simulink model "eml_hdl_design_patterns"  (R2026a)
settings: Solver=FixedStepDiscrete  StopTime=10
InitFcn:
  | errMsg  = ['\n\nThis model is only for demonstration purposes.\n\nPlease do not Simulate or code generate directly from this model. \n\nBefore generating code from this model please do copy the relevant blocks of interest from this model to a new model, place them in a subsystem, build a valid test bench around them.\n\nPlease refer to the example model ''eml_hdl_incrementer'' or HDLCoder documentation'];
  | error(sprintf(errMsg));
undefined symbols (not defined in the file or in its folder): C, gain_val, init_val, lower_limit, maxWordLength, thresh, upper_limit
libraries: simulink x2
(part 1 of 5)
settings Model: FPTRunName=Active  ExtModeAutoUpdateStatusClock=off  Creator=The MathWorks, Inc.  LastModifiedBy=The MathWorks, Inc.
settings SolverCC: InsertRTBMode=Auto
settings OptimizationCC: ConditionallyExecuteInputs=off  InitFltsAndDblsToZero=on  EfficientMapNaN2IntZero=off
settings DebuggingCC: AlgebraicLoopMsg=error  UnderspecifiedInitializationDetection=Classic  SingleTaskRateTransMsg=error
settings HardwareCC: ProdHWDeviceType=ASIC/FPGA  ProdEqTarget=off
settings GRTTargetCC: TargetFcnLib=ansi_tfl_tmw_new.mat  CombineOutputUpdateFcns=off  GRTInterface=on

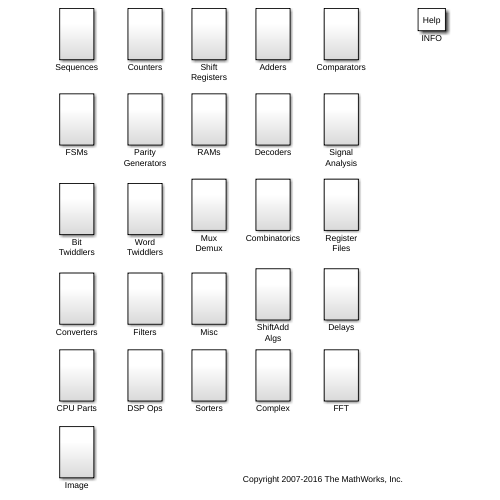
[thumbnail: Simulink's stored preview of the top-level diagram]
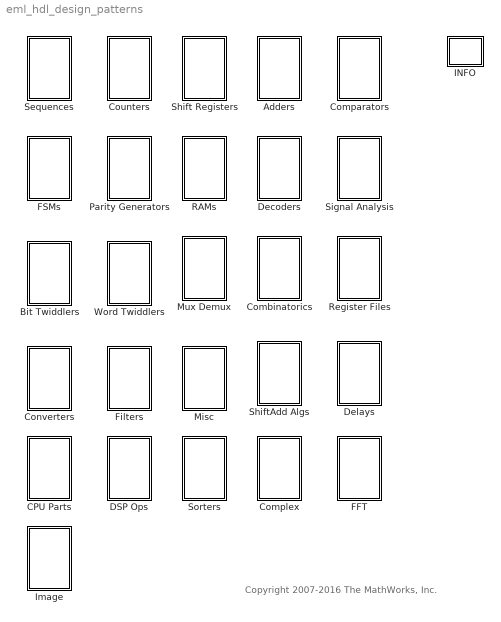
== system eml_hdl_design_patterns ==
  note: Copyright 2007-2016 The MathWorks, Inc.
  Adders : Subsystem
  Bit Twiddlers : Subsystem
  CPU Parts : Subsystem
  Combinatorics : Subsystem
  Comparators : Subsystem
  Complex : Subsystem
  Converters : Subsystem
  Counters : Subsystem
  DSP Ops : Subsystem
  Decoders : Subsystem
  Delays : Subsystem
  FFT : Subsystem
  FSMs : Subsystem
  Filters : Subsystem
  INFO : Subsystem
      settings: OpenFcn=helpview(fullfile (docroot,'toolbox','hdlcoder','ug','hdlcoder_ug.map'), 'slhdlcoder_eml_design_patterns');
      mask Display: disp('Help')
  Image : Subsystem
  Misc : Subsystem
  Mux Demux : Subsystem
  Parity Generators : Subsystem
  RAMs : Subsystem
  Register Files : Subsystem
  Sequences : Subsystem
  Shift Registers : Subsystem
  ShiftAdd Algs : Subsystem
  Signal Analysis : Subsystem
  Sorters : Subsystem
  Word Twiddlers : Subsystem

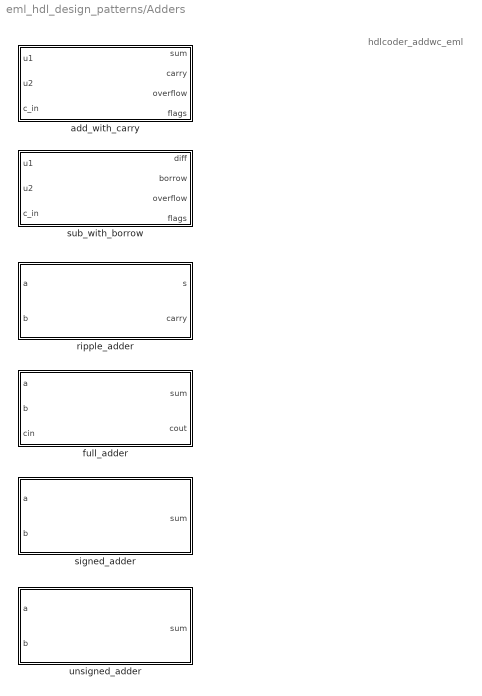
== system eml_hdl_design_patterns/Adders ==
  note: hdlcoder_addwc_eml
  add_with_carry : MATLAB Function  TreatAsAtomicUnit=on
  full_adder : MATLAB Function  TreatAsAtomicUnit=on
  ripple_adder : MATLAB Function  TreatAsAtomicUnit=on
  signed_adder : MATLAB Function  TreatAsAtomicUnit=on
  sub_with_borrow : MATLAB Function  TreatAsAtomicUnit=on
  unsigned_adder : MATLAB Function  TreatAsAtomicUnit=on

== system eml_hdl_design_patterns/Bit Twiddlers ==
  note: hdlcoder_bitops_eml
  note: hdlcoder_int2bits_bits2int
  hdl_bit_ops : MATLAB Function  TreatAsAtomicUnit=on

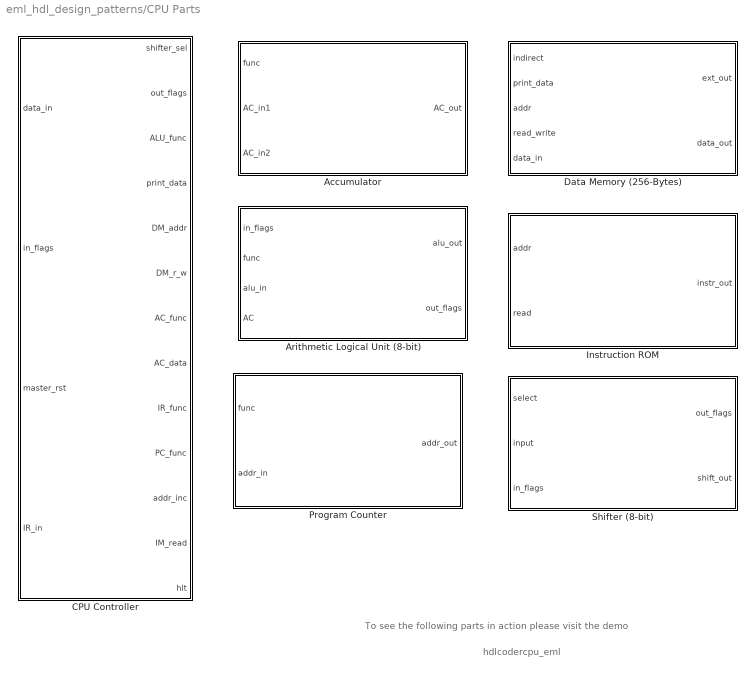
== system eml_hdl_design_patterns/CPU Parts ==
  note: To see the following parts in action please visit the demo
  note: hdlcodercpu_eml
  Accumulator : MATLAB Function  TreatAsAtomicUnit=on
  Arithmetic Logical Unit (8-bit) : MATLAB Function  TreatAsAtomicUnit=on
  CPU Controller : MATLAB Function  TreatAsAtomicUnit=on
  Data Memory (256-Bytes) : MATLAB Function  TreatAsAtomicUnit=on
  Instruction ROM : MATLAB Function  TreatAsAtomicUnit=on
  Program Counter : MATLAB Function  TreatAsAtomicUnit=on
  Shifter (8-bit) : MATLAB Function  TreatAsAtomicUnit=on

== system eml_hdl_design_patterns/Combinatorics ==
  count_ones_blk : MATLAB Function  TreatAsAtomicUnit=on
  eml_expr : MATLAB Function  TreatAsAtomicUnit=on
  hierarchical_mimoparts : Subsystem
  monolithic_mimoparts : MATLAB Function  TreatAsAtomicUnit=on
  pow2Test : MATLAB Function  TreatAsAtomicUnit=on

== system eml_hdl_design_patterns/Comparators ==
  eml_linear_min : MATLAB Function  TreatAsAtomicUnit=on
  eml_tree_min : MATLAB Function  TreatAsAtomicUnit=on

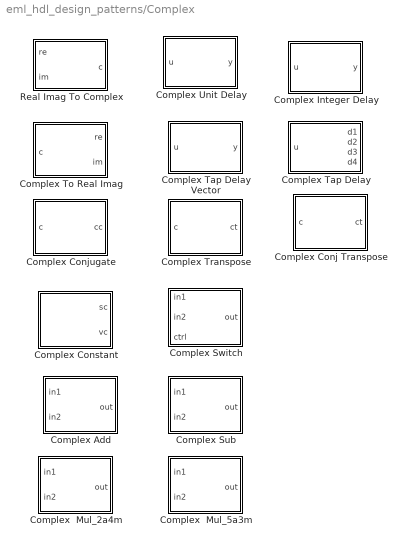
== system eml_hdl_design_patterns/Complex ==
  Complex  Mul_2a4m : MATLAB Function  TreatAsAtomicUnit=on
  Complex  Mul_5a3m : MATLAB Function  TreatAsAtomicUnit=on
  Complex Add : MATLAB Function  TreatAsAtomicUnit=on
  Complex Conj Transpose : MATLAB Function  TreatAsAtomicUnit=on
  Complex Conjugate : MATLAB Function  TreatAsAtomicUnit=on
  Complex Constant : MATLAB Function  TreatAsAtomicUnit=on
  Complex Integer Delay : MATLAB Function  TreatAsAtomicUnit=on
  Complex Sub : MATLAB Function  TreatAsAtomicUnit=on
  Complex Switch : MATLAB Function  TreatAsAtomicUnit=on
  Complex Tap Delay : MATLAB Function  TreatAsAtomicUnit=on
  Complex Tap Delay Vector : MATLAB Function  TreatAsAtomicUnit=on
  Complex To Real Imag : MATLAB Function  TreatAsAtomicUnit=on
  Complex Transpose : MATLAB Function  TreatAsAtomicUnit=on
  Complex Unit Delay : MATLAB Function  TreatAsAtomicUnit=on
  Real Imag To Complex : MATLAB Function  TreatAsAtomicUnit=on

== system eml_hdl_design_patterns/Converters ==
  gray2bin_blk : MATLAB Function  TreatAsAtomicUnit=on

== system eml_hdl_design_patterns/Counters ==
  note: hdlcoder_counters_eml
  counter_clear : MATLAB Function  TreatAsAtomicUnit=on
  counter_mod3 : MATLAB Function  TreatAsAtomicUnit=on
  counter_preset_clear : MATLAB Function  TreatAsAtomicUnit=on
  counter_up_down_enable : MATLAB Function  TreatAsAtomicUnit=on
  gray_counter : MATLAB Function  TreatAsAtomicUnit=on
  johnson_counter : MATLAB Function  TreatAsAtomicUnit=on

== system eml_hdl_design_patterns/DSP Ops ==
  dsp_fold : MATLAB Function  TreatAsAtomicUnit=on
  dsp_scale : MATLAB Function  TreatAsAtomicUnit=on
  dsp_shift : MATLAB Function  TreatAsAtomicUnit=on
  dsp_sum : MATLAB Function  TreatAsAtomicUnit=on

== system eml_hdl_design_patterns/Decoders ==
  note: hdlcoderviterbi2
  note: To see the following parts in action please visit the demo
  decoder_2_by_4 : MATLAB Function  TreatAsAtomicUnit=on
  decoder_n_bit : MATLAB Function  TreatAsAtomicUnit=on
  hierarchical_viterbi : Subsystem
      mask Display: disp('Fixed Point\nViterbi Decoder\nUsing Multiple\nMATLAB Function Blocks');
  monlithic_viterbi : MATLAB Function  TreatAsAtomicUnit=on

== system eml_hdl_design_patterns/Delays ==
  note: hdlcoder_delays_eml
  Integer Delay : MATLAB Function  TreatAsAtomicUnit=on
  Tap Delay : MATLAB Function  TreatAsAtomicUnit=on
  Tap Delay Vector : MATLAB Function  TreatAsAtomicUnit=on
  Unit Delay : MATLAB Function  TreatAsAtomicUnit=on

== system eml_hdl_design_patterns/FFT ==
  note: hdlcoder_fft32_eml
  note: hdlcoder_ofdm_fft_eml
  fft_blk : MATLAB Function  TreatAsAtomicUnit=on

== system eml_hdl_design_patterns/FSMs ==
  note: hdlcoder_fsm_eml
  detect even 1's and odd 0's : MATLAB Function  TreatAsAtomicUnit=on
  mealy_fsm : MATLAB Function  TreatAsAtomicUnit=on
  moore_fsm : MATLAB Function  TreatAsAtomicUnit=on

== system eml_hdl_design_patterns/Filters ==
  lms : MATLAB Function  TreatAsAtomicUnit=on
  sfir_pipelined : MATLAB Function  TreatAsAtomicUnit=on
  symmetric_fir : MATLAB Function  TreatAsAtomicUnit=on

== system eml_hdl_design_patterns/INFO ==
  note: Double Click on the subsystem
      | marked "Help" at the top level
      | to go to the doc page for this model
  note: This model is only for demonstration purposes.
      |
      | It illustrates the power of MATLAB Function Block
      | support in HDLCoder.
      |
      | It shows how to concisely represent common algorithmic
      | operations in ASIC/FPGA applications.
      |
      | Before simulating or code generating from this
      | please copy the relevant blocks from this model to
      | a new model, place them in a subsystem, build
      | a test bench around them with valid inputs.

== system eml_hdl_design_patterns/Image ==
  sobel_edge_behavioral : MATLAB Function  TreatAsAtomicUnit=on
  sobel_edge_serial_pipelined : MATLAB Function  TreatAsAtomicUnit=on
  sobel_edge_serial_pipelined_RAM_mapped : MATLAB Function  TreatAsAtomicUnit=on

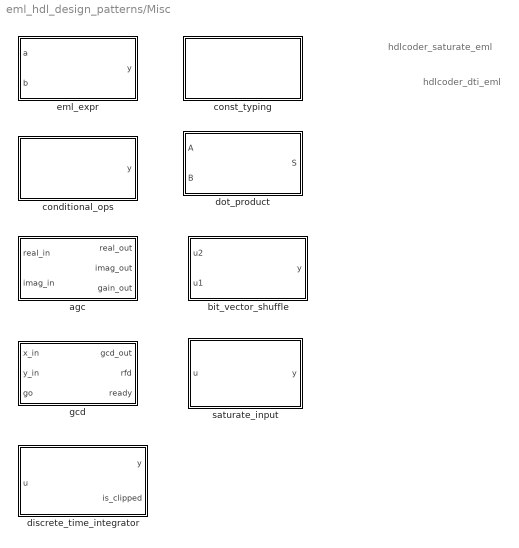
== system eml_hdl_design_patterns/Misc ==
  note: hdlcoder_saturate_eml
  note: hdlcoder_dti_eml
  agc : MATLAB Function  TreatAsAtomicUnit=on
  bit_vector_shuffle : MATLAB Function  TreatAsAtomicUnit=on
  conditional_ops : MATLAB Function  TreatAsAtomicUnit=on
  const_typing : Subsystem
  discrete_time_integrator : MATLAB Function  TreatAsAtomicUnit=on
  dot_product : MATLAB Function  TreatAsAtomicUnit=on
  eml_expr : MATLAB Function  TreatAsAtomicUnit=on
  gcd : MATLAB Function  TreatAsAtomicUnit=on
  saturate_input : MATLAB Function  TreatAsAtomicUnit=on

== system eml_hdl_design_patterns/Mux Demux ==
  demux_using_for_blk : MATLAB Function  TreatAsAtomicUnit=on

== system eml_hdl_design_patterns/Parity Generators ==
  xor_parity_blk : MATLAB Function  TreatAsAtomicUnit=on

== system eml_hdl_design_patterns/RAMs ==
  line_buffer_RAM : MATLAB Function  TreatAsAtomicUnit=on
  sobel_edge_serial_pipelined_RAM_mapped : MATLAB Function  TreatAsAtomicUnit=on

== system eml_hdl_design_patterns/Register Files ==
  dualport_regfile : MATLAB Function  TreatAsAtomicUnit=on
  singleport_regfile : MATLAB Function  TreatAsAtomicUnit=on
  triport_regfile : MATLAB Function  TreatAsAtomicUnit=on

== system eml_hdl_design_patterns/Sequences ==
  stepseq : MATLAB Function  TreatAsAtomicUnit=on

== system eml_hdl_design_patterns/Shift Registers ==
  shift_reg_1by32 : MATLAB Function  TreatAsAtomicUnit=on
  shift_reg_1by64 : MATLAB Function  TreatAsAtomicUnit=on
  shift_reg_universal : MATLAB Function  TreatAsAtomicUnit=on

== system eml_hdl_design_patterns/ShiftAdd Algs ==
  note: hdlcordic_eml
  cordic : Subsystem

== system eml_hdl_design_patterns/Signal Analysis ==
  conv_input_side : MATLAB Function  TreatAsAtomicUnit=on
  conv_output_side : MATLAB Function  TreatAsAtomicUnit=on

== system eml_hdl_design_patterns/Sorters ==
  bitonic_sort : MATLAB Function  TreatAsAtomicUnit=on
  bubble_sort : MATLAB Function  TreatAsAtomicUnit=on

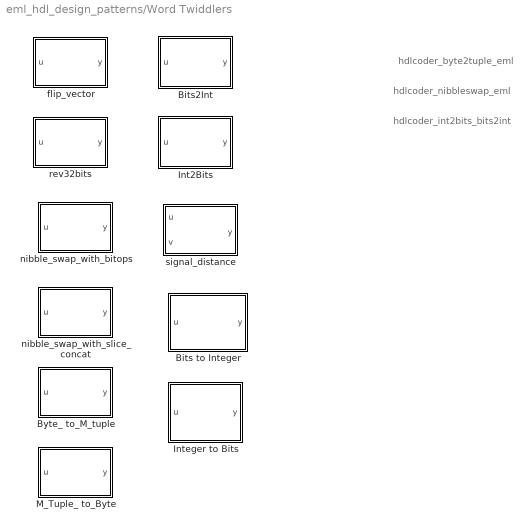
== system eml_hdl_design_patterns/Word Twiddlers ==
  note: hdlcoder_byte2tuple_eml
  note: hdlcoder_nibbleswap_eml
  note: hdlcoder_int2bits_bits2int
  Bits to Integer : MATLAB Function  TreatAsAtomicUnit=on
  Bits2Int : MATLAB Function  TreatAsAtomicUnit=on
  Byte_ to_M_tuple : MATLAB Function  TreatAsAtomicUnit=on
  Int2Bits : MATLAB Function  TreatAsAtomicUnit=on
  Integer to Bits : Subsystem  mask{maxWordLength=maxWordLength}
      mask prompts: maxWordLength "Maximum Word Length"
      mask Display: disp('Integer to Bits')
  M_Tuple_ to_Byte : MATLAB Function  TreatAsAtomicUnit=on
  flip_vector : MATLAB Function  TreatAsAtomicUnit=on
  nibble_swap_with_bitops : MATLAB Function  TreatAsAtomicUnit=on
  nibble_swap_with_slice_concat : MATLAB Function  TreatAsAtomicUnit=on
  rev32bits : MATLAB Function  TreatAsAtomicUnit=on
  signal_distance : MATLAB Function  TreatAsAtomicUnit=on

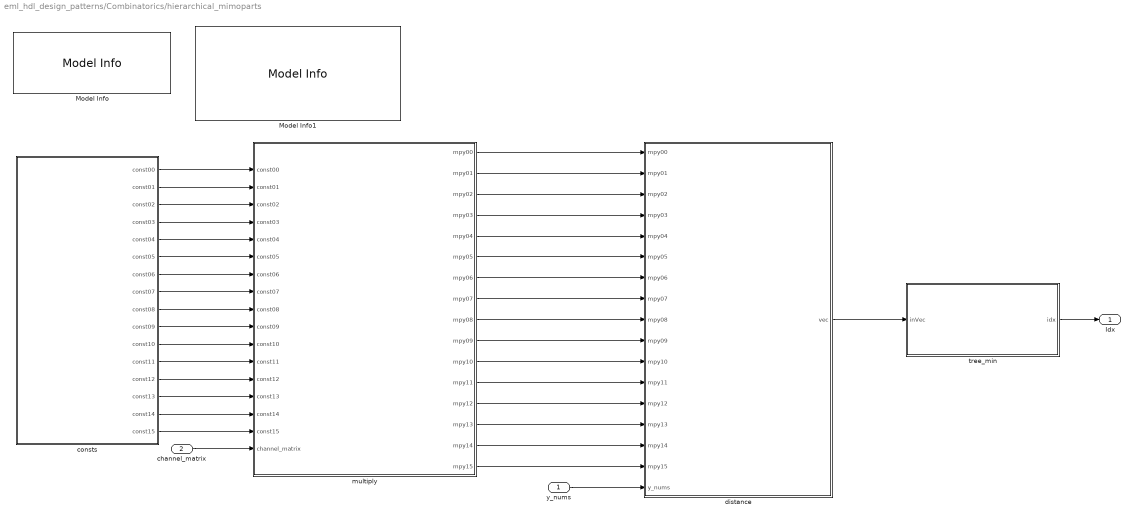
== system eml_hdl_design_patterns/Combinatorics/hierarchical_mimoparts ==
  y_nums : Inport
  channel_matrix : Inport  Port=2
  Model Info : simulink/Model-Wide Utilities/Model Info  Frame=on  DisplayStringWithTags=|  HorizontalTextAlignment=Center  LeftAlignmentValue=0.5
      | This model illustrates some of the
      | key pieces of a MIMO decoder, but
      | is meant only for educational value
      | at this time.
  Model Info1 : simulink/Model-Wide Utilities/Model Info  Frame=on  DisplayStringWithTags=|  HorizontalTextAlignment=Left  LeftAlignmentValue=0.02
      | Key MATLAB Function Block features used in this example:
      | 
      | 1. Creating vector constants
      | 2. Using 'SpecifyPrecision' option in fimath
      | 3. Indexing of vector operands
      | 4. Transpose operations
      | 5. Elementwise product operations
      | 6. Sum of elements operation using sum input
      | 7. Tree min function implementation
      | 8. Vector ports
  consts : MATLAB Function  TreatAsAtomicUnit=on
  distance : MATLAB Function  TreatAsAtomicUnit=on
  multiply : MATLAB Function  TreatAsAtomicUnit=on
  tree_min : MATLAB Function  TreatAsAtomicUnit=on
  Idx : Outport
  wires:
  consts/1(const00) -> multiply/1(const00)
  consts/2(const01) -> multiply/2(const01)
  consts/3(const02) -> multiply/3(const02)
  consts/4(const03) -> multiply/4(const03)
  consts/5(const04) -> multiply/5(const04)
  consts/6(const05) -> multiply/6(const05)
  consts/7(const06) -> multiply/7(const06)
  consts/8(const07) -> multiply/8(const07)
  consts/9(const08) -> multiply/9(const08)
  consts/10(const09) -> multiply/10(const09)
  consts/11(const10) -> multiply/11(const10)
  consts/12(const11) -> multiply/12(const11)
  consts/13(const12) -> multiply/13(const12)
  consts/14(const13) -> multiply/14(const13)
  consts/15(const14) -> multiply/15(const14)
  consts/16(const15) -> multiply/16(const15)
  distance/1(vec) -> tree_min/1(inVec)
  channel_matrix/1 -> multiply/17(channel_matrix)
  multiply/1(mpy00) -> distance/1(mpy00)
  multiply/2(mpy01) -> distance/2(mpy01)
  multiply/3(mpy02) -> distance/3(mpy02)
  multiply/4(mpy03) -> distance/4(mpy03)
  multiply/5(mpy04) -> distance/5(mpy04)
  multiply/6(mpy05) -> distance/6(mpy05)
  multiply/7(mpy06) -> distance/7(mpy06)
  multiply/8(mpy07) -> distance/8(mpy07)
  multiply/9(mpy08) -> distance/9(mpy08)
  multiply/10(mpy09) -> distance/10(mpy09)
  multiply/11(mpy10) -> distance/11(mpy10)
  multiply/12(mpy11) -> distance/12(mpy11)
  multiply/13(mpy12) -> distance/13(mpy12)
  multiply/14(mpy13) -> distance/14(mpy13)
  multiply/15(mpy14) -> distance/15(mpy14)
  multiply/16(mpy15) -> distance/16(mpy15)
  y_nums/1 -> distance/17(y_nums)
  tree_min/1(idx) -> Idx/1

== system eml_hdl_design_patterns/Decoders/hierarchical_viterbi ==
  In1 : Inport  OutDataTypeStr=fixdt(1, 6, 3)  PortDimensions=[2 1]  SampleTime=[10 1]
  BMU1 : MATLAB Function  TreatAsAtomicUnit=on
  PMU1 : Subsystem
  TBU1 : MATLAB Function  TreatAsAtomicUnit=on
  y1 : Outport
  wires:
  TBU1/1(y) -> y1/1
  BMU1/1(bm) -> PMU1/1(bm)
  PMU1/1(dec) -> TBU1/1(dec)
  PMU1/2(index) -> TBU1/2(index)
  In1/1 -> BMU1/1(u)

== system eml_hdl_design_patterns/Misc/const_typing ==
  typed : MATLAB Function  TreatAsAtomicUnit=on
  untyped : MATLAB Function  TreatAsAtomicUnit=on

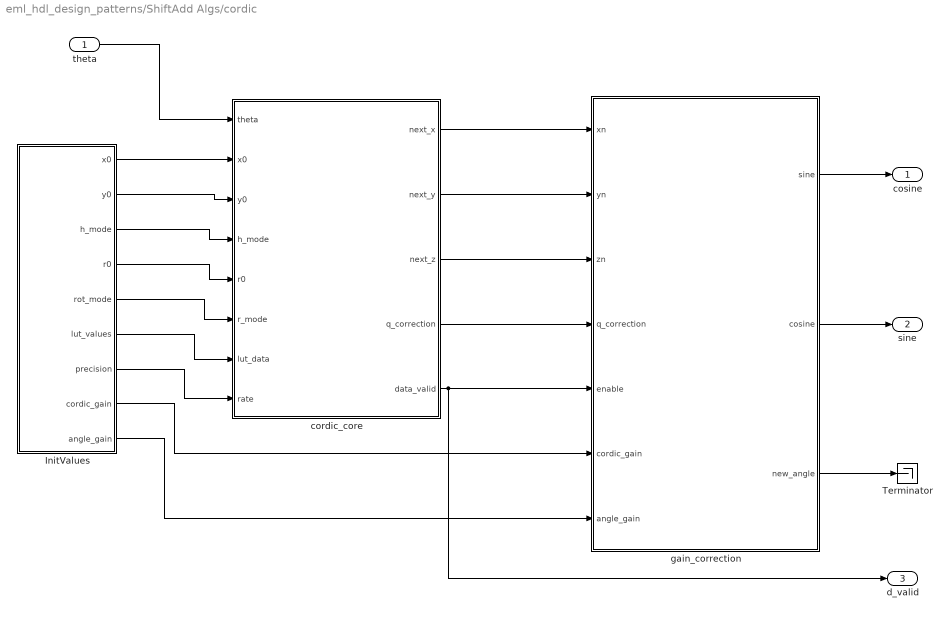
== system eml_hdl_design_patterns/ShiftAdd Algs/cordic ==
  theta : Inport
  InitValues : Subsystem
  Terminator : Terminator
  cordic_core : Subsystem
  gain_correction : MATLAB Function  TreatAsAtomicUnit=on
  cosine : Outport
  sine : Outport  Port=2
  d_valid : Outport  Port=3
  wires:
  gain_correction/1(sine) -> cosine/1
  gain_correction/2(cosine) -> sine/1
  gain_correction/3(new_angle) -> Terminator/1
  cordic_core/1(next_x) -> gain_correction/1(xn)
  cordic_core/2(next_y) -> gain_correction/2(yn)
  cordic_core/3(next_z) -> gain_correction/3(zn)
  cordic_core/4(q_correction) -> gain_correction/4(q_correction)
  cordic_core/5(data_valid) -> gain_correction/5(enable), d_valid/1
  InitValues/8(cordic_gain) -> gain_correction/6(cordic_gain)
  InitValues/9(angle_gain) -> gain_correction/7(angle_gain)
  theta/1 -> cordic_core/1(theta)
  InitValues/1(x0) -> cordic_core/2(x0)
  InitValues/2(y0) -> cordic_core/3(y0)
  InitValues/3(h_mode) -> cordic_core/4(h_mode)
  InitValues/4(r0) -> cordic_core/5(r0)
  InitValues/5(rot_mode) -> cordic_core/6(r_mode)
  InitValues/6(lut_values) -> cordic_core/7(lut_data)
  InitValues/7(precision) -> cordic_core/8(rate)

== system eml_hdl_design_patterns/Word Twiddlers/Integer to Bits ==
  u : Inport
  MATLAB Function : MATLAB Function  TreatAsAtomicUnit=on
  y : Outport
  wires:
  MATLAB Function/1(y) -> y/1
  u/1 -> MATLAB Function/1(u)

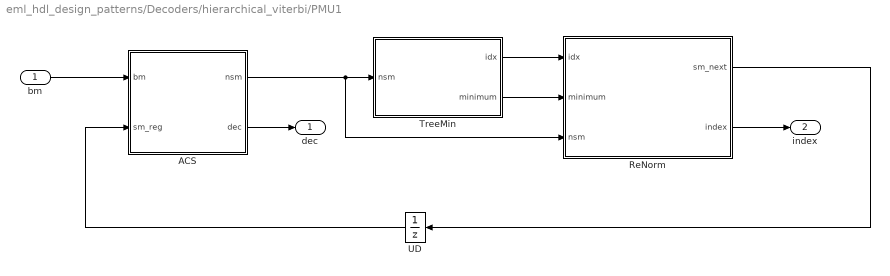
== system eml_hdl_design_patterns/Decoders/hierarchical_viterbi/PMU1 ==
  bm : Inport
  ACS : MATLAB Function  TreatAsAtomicUnit=on
  ReNorm : MATLAB Function  TreatAsAtomicUnit=on
  TreeMin : MATLAB Function  TreatAsAtomicUnit=on
  UD : UnitDelay  SampleTime=-1
  dec : Outport
  index : Outport  Port=2
  wires:
  bm/1 -> ACS/1(bm)
  ACS/1(nsm) -> TreeMin/1(nsm), ReNorm/3(nsm)
  TreeMin/1(idx) -> ReNorm/1(idx)
  TreeMin/2(minimum) -> ReNorm/2(minimum)
  ACS/2(dec) -> dec/1
  ReNorm/1(sm_next) -> UD/1
  ReNorm/2(index) -> index/1
  UD/1 -> ACS/2(sm_reg)

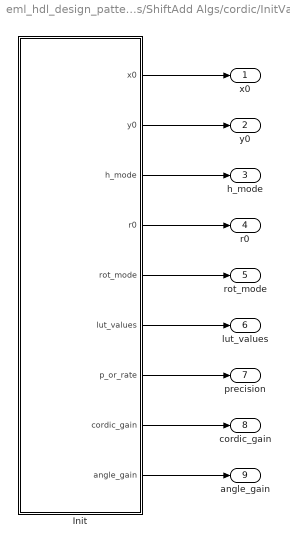
== system eml_hdl_design_patterns/ShiftAdd Algs/cordic/InitValues ==
  Init : MATLAB Function  TreatAsAtomicUnit=on
  x0 : Outport
  y0 : Outport  Port=2
  h_mode : Outport  Port=3
  r0 : Outport  Port=4
  rot_mode : Outport  Port=5
  lut_values : Outport  Port=6
  precision : Outport  Port=7
  cordic_gain : Outport  Port=8
  angle_gain : Outport  Port=9
  wires:
  Init/1(x0) -> x0/1
  Init/2(y0) -> y0/1
  Init/3(h_mode) -> h_mode/1
  Init/4(r0) -> r0/1
  Init/5(rot_mode) -> rot_mode/1
  Init/6(lut_values) -> lut_values/1
  Init/7(p_or_rate) -> precision/1
  Init/8(cordic_gain) -> cordic_gain/1
  Init/9(angle_gain) -> angle_gain/1

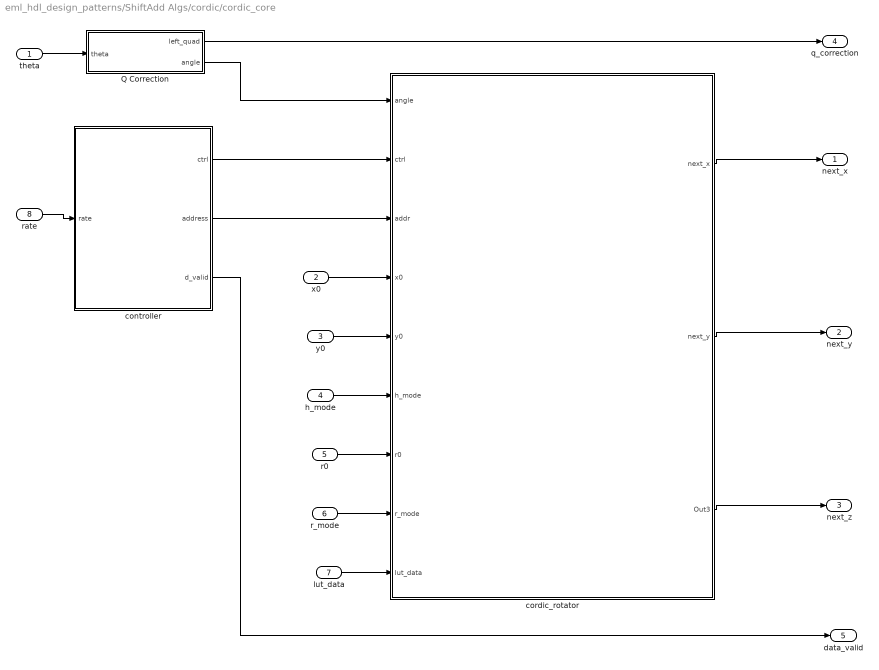
== system eml_hdl_design_patterns/ShiftAdd Algs/cordic/cordic_core ==
  theta : Inport
  x0 : Inport  Port=2
  y0 : Inport  Port=3
  h_mode : Inport  Port=4
  r0 : Inport  Port=5
  r_mode : Inport  Port=6
  lut_data : Inport  Port=7
  rate : Inport  Port=8
  Q Correction : MATLAB Function  TreatAsAtomicUnit=on
  controller : MATLAB Function  TreatAsAtomicUnit=on
  cordic_rotator : Subsystem
  next_x : Outport
  next_y : Outport  Port=2
  next_z : Outport  Port=3
  q_correction : Outport  Port=4
  data_valid : Outport  Port=5
  wires:
  controller/3(d_valid) -> data_valid/1
  rate/1 -> controller/1(rate)
  cordic_rotator/2(next_y) -> next_y/1
  cordic_rotator/1(next_x) -> next_x/1
  cordic_rotator/3(Out3) -> next_z/1
  theta/1 -> Q Correction/1(theta)
  Q Correction/1(left_quad) -> q_correction/1
  x0/1 -> cordic_rotator/4(x0)
  h_mode/1 -> cordic_rotator/6(h_mode)
  r0/1 -> cordic_rotator/7(r0)
  r_mode/1 -> cordic_rotator/8(r_mode)
  lut_data/1 -> cordic_rotator/9(lut_data)
  y0/1 -> cordic_rotator/5(y0)
  Q Correction/2(angle) -> cordic_rotator/1(angle)
  controller/1(ctrl) -> cordic_rotator/2(ctrl)
  controller/2(address) -> cordic_rotator/3(addr)

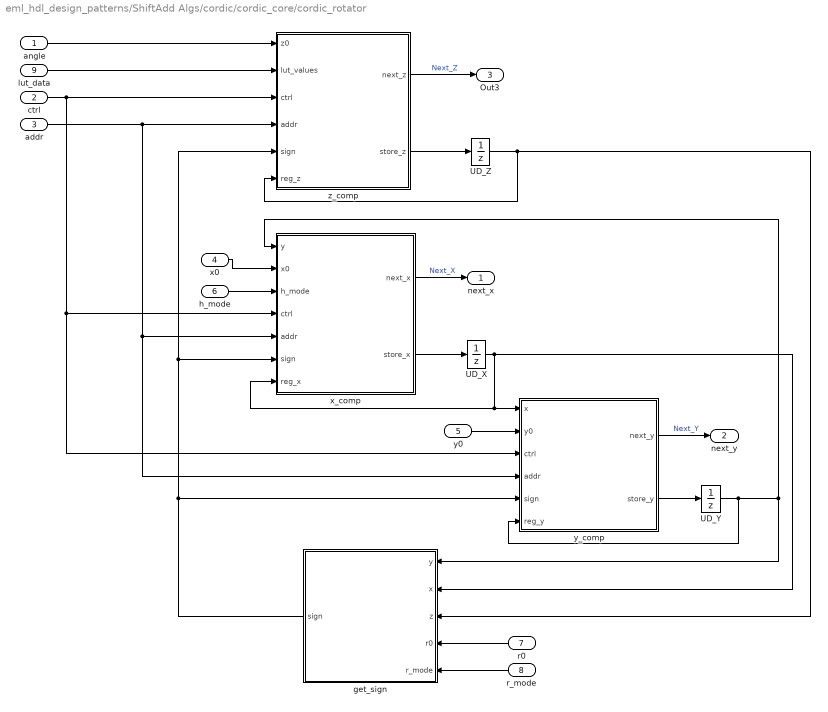
== system eml_hdl_design_patterns/ShiftAdd Algs/cordic/cordic_core/cordic_rotator ==
  angle : Inport
  ctrl : Inport  Port=2
  addr : Inport  Port=3
  x0 : Inport  Port=4
  y0 : Inport  Port=5
  h_mode : Inport  Port=6
  r0 : Inport  Port=7
  r_mode : Inport  Port=8
  lut_data : Inport  Port=9
  UD_X : UnitDelay  SampleTime=-1
  UD_Y : UnitDelay  SampleTime=-1
  UD_Z : UnitDelay  SampleTime=-1
  get_sign : MATLAB Function  TreatAsAtomicUnit=on
  x_comp : MATLAB Function  TreatAsAtomicUnit=on
  y_comp : MATLAB Function  TreatAsAtomicUnit=on
  z_comp : MATLAB Function  TreatAsAtomicUnit=on
  next_x : Outport
  next_y : Outport  Port=2
  Out3 : Outport  Port=3
  wires:
  r_mode/1 -> get_sign/5(r_mode)
  r0/1 -> get_sign/4(r0)
  addr/1 -> y_comp/4(addr), x_comp/5(addr), z_comp/4(addr)
  ctrl/1 -> y_comp/3(ctrl), x_comp/4(ctrl), z_comp/3(ctrl)
  lut_data/1 -> z_comp/2(lut_values)
  y0/1 -> y_comp/2(y0)
  h_mode/1 -> x_comp/3(h_mode)
  x0/1 -> x_comp/2(x0)
  y_comp/2(store_y) -> UD_Y/1
  get_sign/1(sign) -> y_comp/5(sign), z_comp/5(sign), x_comp/6(sign)
  UD_Z/1 -> z_comp/6(reg_z), get_sign/3(z)
  UD_Y/1 -> y_comp/6(reg_y), get_sign/1(y), x_comp/1(y)
  UD_X/1 -> y_comp/1(x), x_comp/7(reg_x), get_sign/2(x)
  x_comp/2(store_x) -> UD_X/1
  z_comp/2(store_z) -> UD_Z/1
  angle/1 -> z_comp/1(z0)
  x_comp/1(next_x) -> next_x/1  "Next_X"
  y_comp/1(next_y) -> next_y/1  "Next_Y"
  z_comp/1(next_z) -> Out3/1  "Next_Z"

== matlab function eml_hdl_design_patterns/Complex/Complex  Mul_2a4m ==
  settings: fimath=|
      | fimath(...
      | 'RoundMode', 'floor',...
      | 'OverflowMode', 'wrap',...
      | 'ProductMode', 'FullPrecision', 'ProductWordLength', 32,...
      | 'SumMode', 'FullPrecision', 'SumWordLength', 32,...
      | 'CastBeforeSum', true)
  data: out output; in1 input fixdt(1,14,2); in2 input fixdt(1,14,2)
function out = fcn(in1, in2)
% Compute Multiply
%
%  out_re = in1_re * in2_re - in1_im * in2_im
%  out_im = in1_re * in2_im + in1_im * in2_re
%
% For fixed point inputs 'SumMode' and 'ProductMode' options on the 
% block fimath decides the sum and product semantics in the above equations. 
%
% In this example SumMode and ProductMode are set to FullPrecision 
% which is optimal for HDLCodegen
%
% The default complex multiplication operator uses 2adders and 4multipliers
% shown in the above equations.


f = fimath(in1);
nt = numerictype(in1);

out = fi(in1*in2, nt, f);

== matlab function eml_hdl_design_patterns/Complex/Complex  Mul_5a3m ==
  settings: fimath=|
      | fimath(...
      | 'RoundMode', 'floor',...
      | 'OverflowMode', 'wrap',...
      | 'ProductMode', 'FullPrecision', 'ProductWordLength', 32,...
      | 'SumMode', 'FullPrecision', 'SumWordLength', 32,...
      | 'CastBeforeSum', true)
  data: out output; in1 input; in2 input
function out = fcn(in1, in2)
% Compute Complex Multiply
% 
% The canonical definition of complex multiplication is:
%
%  out_re = in1_re * in2_re - in1_im * in2_im
%  out_im = in1_re * in2_im + in1_im * in2_re
%
% This definition uses 2 adders and 4 multipliers, as shown above.
%
% However, algebraic manipiulation of these equations results in another pair of
% equations that requires only 3 multipliers, while requiring 5 adders. This
% tradeoff results in reduced area consumption for complex multiplication.
%
%  (a + bi) * (c + di) ==> e + fi
%
%    where
%
%  e = (a + b)*(c - d) - b*c + a*d
%  f = b*c + a*d
%
% For fixed point inputs, the 'SumMode' and 'ProductMode' options on the 
% block fimath decide the sum and product semantics for fixed point calculations.
%
% In this example, SumMode and ProductMode are set to FullPrecision, which is
% optimal for HDL code generation.

fm = fimath(in1);
nt = numerictype(in1);

a = real(in1);
b = imag(in1);

c = real(in2);
d = imag(in2);

bc = fi(b .* c, nt, fm);
ad = fi(a .* d, nt, fm);

% Compute the real part
e = fi((a + b) .* (c - d) - bc + ad, nt, fm);
% Compute the imaginary part
f = fi(bc + ad, nt, fm);

out = complex(e, f);
end

== matlab function eml_hdl_design_patterns/Delays/Integer Delay ==
  settings: fimath=|
      | fimath(...
      | 'RoundMode', 'floor',...
      | 'OverflowMode', 'wrap',...
      | 'ProductMode', 'FullPrecision', 'ProductWordLength', 32,...
      | 'SumMode', 'FullPrecision', 'SumWordLength', 32,...
      | 'CastBeforeSum', true)
  data: u input; y output; N parameter
function y = fcn(u, N)

% The Integer Delay block delays its input by N sample periods. 
% The block accepts one input and generates one output, both of which
% can be scalar or vector. If the input is a vector, all elements of the 
% vector are delayed by the same sample period.

% In this example N is hardwired as 4; This function behaves as Integer 
% delay block and delays inputs by 4 sample hits.

persistent u_d;
if isempty(u_d)
	% defines initial value driven by integer delay 
    % from time step 0 to time step N-1
    u_d = fi(zeros(1,N), numerictype(u), fimath(u));
end

y = u_d(N);

u_d = [u, u_d(1:N-1)];

== matlab function eml_hdl_design_patterns/Counters/johnson_counter ==
  settings: fimath=|
      | fimath(...
      | 'RoundMode', 'floor',...
      | 'OverflowMode', 'saturate',...
      | 'ProductMode', 'FullPrecision', 'ProductWordLength', 32,...
      | 'SumMode', 'FullPrecision', 'SumWordLength', 32,...
      | 'CastBeforeSum', true)
  data: enable input boolean; count output fixdt(0,4,0) size=1
function count = fcn(enable)

% A johnson counter is a circular shift register that feeds the LSB with
% the inverted MSB.  It generates a pattern like
% 0000
% 0001
% 0011
% 0111
% 1111
% 1110
% 1100
% 1000
% 0000
% 0001

% This counter is configured to rollover.  If this is not desirable,
% set result_fm 'OverflowMode' to 'saturate'.

result_nt = numerictype(0,4,0);
result_fm = fimath('OverflowMode', 'wrap', 'RoundMode', 'floor');

persistent count_reg;

if isempty(count_reg)
    count_reg = fi(0, result_nt, result_fm);
end

% Assign the output even when we're not enabled.
count = count_reg;

if enable
   oldmsb = getmsb(count_reg);
   count_reg = bitsll(count_reg, 1);   
   count_reg = bitset(count_reg, 1, ~uint8(oldmsb));
end

== matlab function eml_hdl_design_patterns/Delays/Tap Delay Vector ==
  settings: fimath=|
      | fimath(...
      | 'RoundMode', 'floor',...
      | 'OverflowMode', 'wrap',...
      | 'ProductMode', 'FullPrecision', 'ProductWordLength', 32,...
      | 'SumMode', 'FullPrecision', 'SumWordLength', 32,...
      | 'CastBeforeSum', true)
  data: u input; y output
function y = fcn(u)
% The Tapped Delay function delays its input by the specified number 
% of sample periods, and outputs all the delayed versions in a vector
% form.

% In this example N is hardwired to 4.

persistent u_d;
if isempty(u_d)
    u_d = fi(zeros(1,4), numerictype(u), fimath(u));
end

y = u_d;

u_d = [u_d(2), u_d(3), u_d(4), u];

== matlab function eml_hdl_design_patterns/Delays/Tap Delay ==
  settings: fimath=|
      | fimath(...
      | 'RoundMode', 'floor',...
      | 'OverflowMode', 'wrap',...
      | 'ProductMode', 'FullPrecision', 'ProductWordLength', 32,...
      | 'SumMode', 'FullPrecision', 'SumWordLength', 32,...
      | 'CastBeforeSum', true)
  data: u input; d1 output; d2 output; d3 output; d4 output
function [d1, d2, d3, d4] = fcn(u)
%The Tapped Delay function delays its input by the specified number 
% of sample periods, and outputs all the delayed versions.

% In this example the number of output taps is hardwired to 4.

persistent u_d;
if isempty(u_d)
    % defines initial value driven by integer delay 
    % from time step 0 to time step N-1
    u_d = fi(zeros(1,4), numerictype(u), fimath(u));
end

d1 = u_d(1);
d2 = u_d(2);
d3 = u_d(3);
d4 = u_d(4);

u_d = [u_d(2:4), u];

== matlab function eml_hdl_design_patterns/Word Twiddlers/Int2Bits ==
  data: u input; y output
function y = fcn(u)
% Converts Integer(8bits) to a 1-D array Bits

y = bitget(u, [8:-1:1])';

== matlab function eml_hdl_design_patterns/Image/sobel_edge_serial_pipelined ==
  settings: fimath=|
      | fimath(...
      | 'RoundMode', 'floor',...
      | 'OverflowMode', 'wrap',...
      | 'ProductMode', 'FullPrecision', 'ProductWordLength', 32,...
      | 'SumMode', 'FullPrecision', 'SumWordLength', 32,...
      | 'CastBeforeSum', true)
  data: u input fixdt(1,9,0); e output; thresh parameter uint8
function e = fcn(u, thresh)
% Pipelined Sobel Edge Detection algorithm on serialized image.

[xfo, yfo] =  filter(u);
xfd = filterdelay12(xfo);
yfd = filterdelay13(yfo);
ax = abs(xfd);
ay = abs(yfd);
t = (ax + ay >= thresh);
e = filterdelay14(t);

end

%%%%%%%%%%%%%%%%%%%%%%%%%%%%%%%%%%%%%%%%%%%%%%%%%%%%%%%%%%%%%%%%%%%%%%%%%%%
% Compute convolution of serialized image data with sobel masks
%%%%%%%%%%%%%%%%%%%%%%%%%%%%%%%%%%%%%%%%%%%%%%%%%%%%%%%%%%%%%%%%%%%%%%%%%%%
function [xfo, yfo] =  filter(u)

lb1 = line_buffer1(u);
lb2 = line_buffer2(lb1);

ud1 = filterdelay1(u);
ud2 = filterdelay2(ud1);

lb1d1 = filterdelay3(lb1);
lb1d2 = filterdelay4(lb1d1);

lb2d1 = filterdelay5(lb2);
lb2d2 = filterdelay6(lb2d1);

xfo = xf(u, ud1, ud2, lb2, lb2d1, lb2d2);
yfo = yf(ud2, u, lb1d2, lb1, lb2d2, lb2);

end

%%%%%%%%%%%%%%%%%%%%%%%%%%%%%%%%%%%%%%%%%%%%%%%%%%%%%%%%%%%%%%%%%%%%%%%%%%%
% Compute x gradient
%%%%%%%%%%%%%%%%%%%%%%%%%%%%%%%%%%%%%%%%%%%%%%%%%%%%%%%%%%%%%%%%%%%%%%%%%%%
function xf_out = xf(u, xd1, xd2, lb2, zd1, zd2)
c2 = fi(2, 1,3,0, fimath(u));

t1 = fi(xd1 * c2, 1,10,0, fimath(u));
a1 = fi(u + t1 + xd2, 1,11,0, fimath(u));
pa1 = filterdelay7(a1);

t1 = fi(zd1 * c2, 1,10,0, fimath(u));
a2 = fi(lb2 + t1 + zd2, 1,11,0, fimath(u));
pa2 = filterdelay8(a2);

xf_out = fi(pa1 - pa2, 1,12,0, fimath(u));

end

%%%%%%%%%%%%%%%%%%%%%%%%%%%%%%%%%%%%%%%%%%%%%%%%%%%%%%%%%%%%%%%%%%%%%%%%%%%
% Compute y gradient
%%%%%%%%%%%%%%%%%%%%%%%%%%%%%%%%%%%%%%%%%%%%%%%%%%%%%%%%%%%%%%%%%%%%%%%%%%%
function yf_out = yf(xd2, u, yd2, lb1, zd2, lb2)
t = fi(xd2 - u, 1,11,0, fimath(u));
pa1 = filterdelay9(t);

t = fi(yd2 - lb1, 1,11,0, fimath(u));
c2 = fi(2, 1,3,0, fimath(u));
a2 = fi(c2 * t, 1,11,0, fimath(u));
pa2 = filterdelay10(a2);

t = fi(zd2 - lb2, 1,11,0, fimath(u));
pa3 = filterdelay11(t);

yf_out = fi(pa1 + pa2 + pa3, 1,13,0, fimath(u));

end

%%%%%%%%%%%%%%%%%%%%%%%%%%%%%%%%%%%%%%%%%%%%%%%%%%%%%%%%%%%%%%%%%%%%%%%%%%%
% Line Buffers %
%%%%%%%%%%%%%%%%%%%%%%%%%%%%%%%%%%%%%%%%%%%%%%%%%%%%%%%%%%%%%%%%%%%%%%%%%%%
function y = line_buffer1(u)
N = 100;
persistent u_d;
if isempty(u_d)
    u_d = fi(zeros(1,N), numerictype(u), fimath(u));
end

y = u_d(N);
u_d = [u, u_d(1:N-1)];
end

function y = line_buffer2(u)
N = 100;
persistent u_d;
if isempty(u_d)
    u_d = fi(zeros(1,N), numerictype(u), fimath(u));
end

y = u_d(N);
u_d = [u, u_d(1:N-1)];
end


%%%%%%%%%%%%%%%%%%%%%%%%%%%%%%%%%%%%%%%%%%%%%%%%%%%%%%%%%%%%%%%%%%%%%%%%%%%
% Filter Delays %
%%%%%%%%%%%%%%%%%%%%%%%%%%%%%%%%%%%%%%%%%%%%%%%%%%%%%%%%%%%%%%%%%%%%%%%%%%%

function y = filterdelay1(u)
persistent u_d;
if isempty(u_d)
    u_d = fi(0, numerictype(u), fimath(u));
end
y = u_d;
u_d = u;
end

function y = filterdelay2(u)
persistent u_d;
if isempty(u_d)
    u_d = fi(0, numerictype(u), fimath(u));
end
y = u_d;
u_d = u;
end

function y = filterdelay3(u)
persistent u_d;
if isempty(u_d)
    u_d = fi(0, numerictype(u), fimath(u));
end
y = u_d;
u_d = u;
end

function y = filterdelay4(u)
persistent u_d;
if isempty(u_d)
    u_d = fi(0, numerictype(u), fimath(u));
end
y = u_d;
u_d = u;
end

function y = filterdelay5(u)
persistent u_d;
if isempty(u_d)
    u_d = fi(0, numerictype(u), fimath(u));
end
y = u_d;
u_d = u;
end

function y = filterdelay6(u)
persistent u_d;
if isempty(u_d)
    u_d = fi(0, numerictype(u), fimath(u));
end
y = u_d;
u_d = u;
end

function y = filterdelay7(u)
persistent u_d;
if isempty(u_d)
    u_d = fi(0, numerictype(u), fimath(u));
end
y = u_d;
u_d = u;
end

function y = filterdelay8(u)
persistent u_d;
if isempty(u_d)
    u_d = fi(0, numerictype(u), fimath(u));
end
y = u_d;
u_d = u;
end

function y = filterdelay9(u)
persistent u_d;
if isempty(u_d)
    u_d = fi(0, numerictype(u), fimath(u));
end
y = u_d;
u_d = u;
end

function y = filterdelay10(u)
persistent u_d;
if isempty(u_d)
    u_d = fi(0, numerictype(u), fimath(u));
end
y = u_d;
u_d = u;
end

function y = filterdelay11(u)
persistent u_d;
if isempty(u_d)
    u_d = fi(0, numerictype(u), fimath(u));
end
y = u_d;
u_d = u;
end

function y = filterdelay12(u)
persistent u_d;
if isempty(u_d)
    u_d = fi(0, numerictype(u), fimath(u));
end
y = u_d;
u_d = u;
end

function y = filterdelay13(u)
persistent u_d;
if isempty(u_d)
    u_d = fi(0, numerictype(u), fimath(u));
end
y = u_d;
u_d = u;
end

function y = filterdelay14(u)
persistent u_d;
if isempty(u_d)
    u_d = false;
end
y = u_d;
u_d = u;
end

== matlab function eml_hdl_design_patterns/Filters/lms ==
  settings: fimath=|
      | fimath(...
      | 'RoundMode', 'Nearest',...
      | 'OverflowMode', 'Saturate',...
      | 'ProductMode', 'KeepLSB', 'ProductWordLength', 32, ...
      | 'SumMode', 'KeepLSB', 'SumWordLength', 32, ...
      | 'CastBeforeSum', true)
  data: input input; y output; desired input; step_size input; reset_weights input
function y = fcn(input, desired, step_size, reset_weights)
% Adaptive Noise Canceler algorithm using Least Mean Square (LMS) filter 
% implemented with a MATLAB Function. 
%
% 'input'  : The signal from Exterior Mic which records the ambient noise.
% 'desired': The signal from Pilot's Mic which includes 
%            original music signal and the noise signal
% 'err_sig': The difference between the 'desired' and the filtered 'input'
%            It represents the estimated music signal (output of this block)
% 
% The LMS filter is trying to retrieve the original music signal ('err_sig') 
% from Pilot's Mic by filtering the Exterior Mic's signal and using it to 
% cancel the noise in Pilot's Mic. The coefficients/weights of the filter 
% are updated(adapted) in realtime based on 'input' and 'err_sig'.

fm = fimath(input);

% register filter coefficients
persistent filter_coefficients;
if isempty(filter_coefficients)
    filter_coefficients = fi(zeros(1, 40), 1, 16, 16, fm);
end

% Variable Filter
% call 'tapped_delay_fcn' function on path to create 40-step tapped delay
delayed_signal = tapped_delay_fcn(input);

% apply filter coefficients 
weight_applied = fi(delayed_signal .* filter_coefficients, 1, 32, 20, fm);

% call 'treesum' function on matlab path to sum up the results
filtered_signal = treesum_fcn(weight_applied);

% Output estimated Original Signal
err_sig = fi(desired - filtered_signal, 1, 16, 13, fm);
y = err_sig;

% Update Weights
% call 'update_weight_fcn' function on matlab path to 
% calculate the new weights
updated_weight = update_weight_fcn(step_size, err_sig, delayed_signal, ...
                                   filter_coefficients, reset_weights);

% update filter coefficients register
filter_coefficients = updated_weight;


function tap_delay = tapped_delay_fcn(input)
% The Tapped Delay function delays its input by the specified number 
% of sample periods, and outputs all the delayed versions in a vector
% form. The output includes current input

% NOTE: To instruct MATLAB Coder to compile an external function, 
% add the following compilation directive or pragma to the function code
%#codegen

persistent u_d;
if isempty(u_d)
    u_d = fi(zeros(1,40), numerictype(input), fimath(input));
end


u_d = [u_d(2:40), input];

tap_delay = u_d;


function y = treesum_fcn(u)
%Implement the 'sum' function without a for-loop
%  y = sum(u);

%  The loop based implementation of 'sum' function is not ideal for 
%  HDL generation and results in a longer critical path. 
%  A tree is more efficient as it results in
%  delay of log2(N) instead of a delay of N delay

%  This implementation shows how to explicitly implement the vector sum in 
%  a tree shape to enable hardware optimizations.

%  The ideal way to code this generically for any length of 'u' is to use 
%  recursion but it is not currently supported by the MATLAB Function Block.


% NOTE: To instruct MATLAB Coder to compile an external function, 
% add the following compilation directive or pragma to the function code
%#eml


% Please note that this implementation is hardwired for a 40tap filter.

%20
level1 = vsum(u);

%10
level2 = vsum(level1);

%5
level3 = vsum(level2);

%3
level4 = vsum(level3);

%2
level5 = vsum(level4);

%1
level6 = vsum(level5);


y = level6;



function output = vsum(input)

nt = numerictype(input);
fm = fimath(input);

nd = numel(input)/2;
vt = input(1:2:end);
    
for i = int32(1:nd)
    k = int32(i*2);
    vt(i) = fi(vt(i) + input(k), nt, fm);
end

output = vt;


function weights = update_weight_fcn(step_size, err_sig, delayed_signal, filter_coefficients, reset_weights)
% This function updates the adaptive filter weights based on LMS algorithm

% NOTE: To instruct MATLAB Coder to compile an external function, 
% add the following compilation directive or pragma to the function code
%#eml

fm = fimath(step_size);

step_sig = fi(step_size .* err_sig, 1, 32, 20, fm);
correction_factor = fi(delayed_signal .* step_sig, 1, 32, 20, fm);
updated_weight = fi(correction_factor + filter_coefficients, 1, 16, 16, fm);

if reset_weights
    weights = fi(zeros(1,40), 1, 16, 16, fm);
else    
    weights = updated_weight;
end

== matlab function eml_hdl_design_patterns/Image/sobel_edge_behavioral ==
  data: u input uint8; e output; ref_thresh parameter uint8
function e = fcn(u, ref_thresh)
% SOBEL EDGE DETECTION
%
% Edges characterize boundaries and are therefore a problem of fundamental 
% importance in image processing. Edges in images are areas with strong 
% intensity contrasts. Edge detecting an image significantly 
% reduces the amount of data and filters out useless information, 
% while preserving the important structural properties in an image. 

% The Sobel operator performs a 2-D spatial gradient measurement on an 
% image. Typically it is used to find the approximate absolute gradient 
% magnitude at each point in an input grayscale image. The Sobel edge 
% detector uses a pair of 3x3 convolution masks, one estimating the 
% gradient in the x-direction (columns) and the other estimating the 
% gradient in the y-direction (rows). A convolution mask is usually much 
% smaller than the actual image. As a result, the mask is slid over the 
% image, manipulating a square of pixels at a time. The actual Sobel 
% masks are shown below

% Note that 'gy' is simply 'gx' rotated 90deg anti clockwise
gx = [-1,  0,  1; 
      -2,  0,  2; 
      -1,  0,  1];
  
gy = [ 1,  2,  1;  
       0,  0,  0; 
      -1, -2, -1];

a1t = abs(conv2(gx, double(u), 'full'));
a2t = abs(conv2(gy, double(u), 'full'));

a1 = a1t(3:end-2, 3:end-2);
a2 = a2t(3:end-2, 3:end-2);

% The masks are designed to respond maximally to edges 
% running vertically and horizontally relative to the pixel grid, 
% one mask for each of the two perpendicular orientations. 
% The masks can be applied separately to the input image, 
% to produce separate measurements of the gradient component 
% in each orientation (call these Gx and Gy). These can then 
% be combined together to find the absolute magnitude of the 
% gradient at each point and the orientation of that gradient. 
% The gradient magnitude is given by
%  |G| = sqrt((gx * u)^2 + (gy * u)^2)

e = sqrt(a1 .* a1 + a2 .* a2) >= ref_thresh;

== matlab function eml_hdl_design_patterns/Image/sobel_edge_serial_pipelined_RAM_mapped ==
  settings: fimath=|
      | fimath(...
      | 'RoundMode', 'floor',...
      | 'OverflowMode', 'wrap',...
      | 'ProductMode', 'FullPrecision', 'ProductWordLength', 32,...
      | 'SumMode', 'FullPrecision', 'SumWordLength', 32,...
      | 'CastBeforeSum', true)
  data: u input fixdt(1,9,0); e output; thresh parameter uint8; C parameter
function e = fcn(u, thresh, C)
% Pipelined Sobel Edge Detection algorithm on serialized image.

[xfo, yfo] =  filter(u, C);
xfd = filterdelay12(xfo);
yfd = filterdelay13(yfo);
ax = abs(xfd);
ay = abs(yfd);
t = (ax + ay >= thresh);
e = filterdelay14(t);

end

%%%%%%%%%%%%%%%%%%%%%%%%%%%%%%%%%%%%%%%%%%%%%%%%%%%%%%%%%%%%%%%%%%%%%%%%%%%
% Compute convolution of serialized image data with sobel masks
%%%%%%%%%%%%%%%%%%%%%%%%%%%%%%%%%%%%%%%%%%%%%%%%%%%%%%%%%%%%%%%%%%%%%%%%%%%
function [xfo, yfo] =  filter(u, Col)

lb1 = line_buffer1(u, Col);
lb2 = line_buffer2(lb1, Col);

ud1 = filterdelay1(u);
ud2 = filterdelay2(ud1);

lb1d1 = filterdelay3(lb1);
lb1d2 = filterdelay4(lb1d1);

lb2d1 = filterdelay5(lb2);
lb2d2 = filterdelay6(lb2d1);

xfo = xf(u, ud1, ud2, lb2, lb2d1, lb2d2);
yfo = yf(ud2, u, lb1d2, lb1, lb2d2, lb2);

end

%%%%%%%%%%%%%%%%%%%%%%%%%%%%%%%%%%%%%%%%%%%%%%%%%%%%%%%%%%%%%%%%%%%%%%%%%%%
% Compute x gradient
%%%%%%%%%%%%%%%%%%%%%%%%%%%%%%%%%%%%%%%%%%%%%%%%%%%%%%%%%%%%%%%%%%%%%%%%%%%
function xf_out = xf(u, xd1, xd2, lb2, zd1, zd2)
c2 = fi(2, 1,3,0, fimath(u));

t1 = fi(xd1 * c2, 1,10,0, fimath(u));
a1 = fi(u + t1 + xd2, 1,11,0, fimath(u));
pa1 = filterdelay7(a1);

t1 = fi(zd1 * c2, 1,10,0, fimath(u));
a2 = fi(lb2 + t1 + zd2, 1,11,0, fimath(u));
pa2 = filterdelay8(a2);

xf_out = fi(pa1 - pa2, 1,12,0, fimath(u));

end

%%%%%%%%%%%%%%%%%%%%%%%%%%%%%%%%%%%%%%%%%%%%%%%%%%%%%%%%%%%%%%%%%%%%%%%%%%%
% Compute y gradient
%%%%%%%%%%%%%%%%%%%%%%%%%%%%%%%%%%%%%%%%%%%%%%%%%%%%%%%%%%%%%%%%%%%%%%%%%%%
function yf_out = yf(xd2, u, yd2, lb1, zd2, lb2)
t = fi(xd2 - u, 1,11,0, fimath(u));
pa1 = filterdelay9(t);

t = fi(yd2 - lb1, 1,11,0, fimath(u));
c2 = fi(2, 1,3,0, fimath(u));
a2 = fi(c2 * t, 1,11,0, fimath(u));
pa2 = filterdelay10(a2);

t = fi(zd2 - lb2, 1,11,0, fimath(u));
pa3 = filterdelay11(t);

yf_out = fi(pa1 + pa2 + pa3, 1,13,0, fimath(u));

end

%%%%%%%%%%%%%%%%%%%%%%%%%%%%%%%%%%%%%%%%%%%%%%%%%%%%%%%%%%%%%%%%%%%%%%%%%%%
% Line Buffers %
%%%%%%%%%%%%%%%%%%%%%%%%%%%%%%%%%%%%%%%%%%%%%%%%%%%%%%%%%%%%%%%%%%%%%%%%%%%
function y = line_buffer1(u, N)
persistent u_d ctr;
if isempty(u_d)
    u_d = fi(zeros(1,N), numerictype(u), fimath(u));
    ctr = uint8(1);
end

y = u_d(ctr);
u_d(ctr) = u;

if ctr == N
    ctr = uint8(1);
else
    ctr = ctr + 1;
end
end

function y = line_buffer2(u, N)
persistent u_d ctr;
if isempty(u_d)
    u_d = fi(zeros(1,N), numerictype(u), fimath(u));
    ctr = uint8(1);
end

y = u_d(ctr);
u_d(ctr) = u;

if ctr == N
    ctr = uint8(1);
else
    ctr = ctr + 1;
end
end


%%%%%%%%%%%%%%%%%%%%%%%%%%%%%%%%%%%%%%%%%%%%%%%%%%%%%%%%%%%%%%%%%%%%%%%%%%%
% Filter Delays %
%%%%%%%%%%%%%%%%%%%%%%%%%%%%%%%%%%%%%%%%%%%%%%%%%%%%%%%%%%%%%%%%%%%%%%%%%%%

function y = filterdelay1(u)
persistent u_d;
if isempty(u_d)
    u_d = fi(0, numerictype(u), fimath(u));
end
y = u_d;
u_d = u;
end

function y = filterdelay2(u)
persistent u_d;
if isempty(u_d)
    u_d = fi(0, numerictype(u), fimath(u));
end
y = u_d;
u_d = u;
end

function y = filterdelay3(u)
persistent u_d;
if isempty(u_d)
    u_d = fi(0, numerictype(u), fimath(u));
end
y = u_d;
u_d = u;
end

function y = filterdelay4(u)
persistent u_d;
if isempty(u_d)
    u_d = fi(0, numerictype(u), fimath(u));
end
y = u_d;
u_d = u;
end

function y = filterdelay5(u)
persistent u_d;
if isempty(u_d)
    u_d = fi(0, numerictype(u), fimath(u));
end
y = u_d;
u_d = u;
end

function y = filterdelay6(u)
persistent u_d;
if isempty(u_d)
    u_d = fi(0, numerictype(u), fimath(u));
end
y = u_d;
u_d = u;
end

function y = filterdelay7(u)
persistent u_d;
if isempty(u_d)
    u_d = fi(0, numerictype(u), fimath(u));
end
y = u_d;
u_d = u;
end

function y = filterdelay8(u)
persistent u_d;
if isempty(u_d)
    u_d = fi(0, numerictype(u), fimath(u));
end
y = u_d;
u_d = u;
end

function y = filterdelay9(u)
persistent u_d;
if isempty(u_d)
    u_d = fi(0, numerictype(u), fimath(u));
end
y = u_d;
u_d = u;
end

function y = filterdelay10(u)
persistent u_d;
if isempty(u_d)
    u_d = fi(0, numerictype(u), fimath(u));
end
y = u_d;
u_d = u;
end

function y = filterdelay11(u)
persistent u_d;
if isempty(u_d)
    u_d = fi(0, numerictype(u), fimath(u));
end
y = u_d;
u_d = u;
end

function y = filterdelay12(u)
persistent u_d;
if isempty(u_d)
    u_d = fi(0, numerictype(u), fimath(u));
end
y = u_d;
u_d = u;
end

function y = filterdelay13(u)
persistent u_d;
if isempty(u_d)
    u_d = fi(0, numerictype(u), fimath(u));
end
y = u_d;
u_d = u;
end

function y = filterdelay14(u)
persistent u_d;
if isempty(u_d)
    u_d = false;
end
y = u_d;
u_d = u;
end

== matlab function eml_hdl_design_patterns/RAMs/line_buffer_RAM ==
  settings: fimath=|
      | fimath(...
      | 'RoundMode', 'floor',...
      | 'OverflowMode', 'wrap',...
      | 'ProductMode', 'FullPrecision', 'ProductWordLength', 32,...
      | 'SumMode', 'FullPrecision', 'SumWordLength', 32,...
      | 'CastBeforeSum', true)
  data: u input fixdt(1,9,0); y output; N parameter uint8
%%%%%%%%%%%%%%%%%%%%%%%%%%%%%%%%%%%%%%%%%%%%%%%%%%%%%%%%%%%%%%%%%%%%%%%%%%%
% Line Buffers %
% There are many ways to implement a line buffer in MATLAB. However, if one
% wants to map the line buffer to block RAMs, the it is essential to
% minimize the number of read/write accesses to the buffer, preferably
% keep it to one read and one write. Below is an implementation of line
% buffer that will get automatically mapped to RAMs, if the
% 'MapPersitstentVarsToRAM' property is set to 'on'. Note that, the input,
% 'N' must be an inferrable constant.
%%%%%%%%%%%%%%%%%%%%%%%%%%%%%%%%%%%%%%%%%%%%%%%%%%%%%%%%%%%%%%%%%%%%%%%%%%%

function y = line_buffer(u, N)
persistent buffer ctr;
if isempty(buffer)
    buffer = fi(zeros(1,N), numerictype(u), fimath(u));
    ctr = uint8(1);
end

y = buffer(ctr);
buffer(ctr) = u;

if ctr == N
    ctr = uint8(1);
else
    ctr = ctr + 1;
end
end

== matlab function eml_hdl_design_patterns/RAMs/sobel_edge_serial_pipelined_RAM_mapped ==
  settings: fimath=|
      | fimath(...
      | 'RoundMode', 'floor',...
      | 'OverflowMode', 'wrap',...
      | 'ProductMode', 'FullPrecision', 'ProductWordLength', 32,...
      | 'SumMode', 'FullPrecision', 'SumWordLength', 32,...
      | 'CastBeforeSum', true)
  data: u input fixdt(1,9,0); e output; thresh parameter uint8; C parameter
function e = fcn(u, thresh, C)
% Pipelined Sobel Edge Detection algorithm on serialized image.

[xfo, yfo] =  filter(u, C);
xfd = filterdelay12(xfo);
yfd = filterdelay13(yfo);
ax = abs(xfd);
ay = abs(yfd);
t = (ax + ay >= thresh);
e = filterdelay14(t);

end

%%%%%%%%%%%%%%%%%%%%%%%%%%%%%%%%%%%%%%%%%%%%%%%%%%%%%%%%%%%%%%%%%%%%%%%%%%%
% Compute convolution of serialized image data with sobel masks
%%%%%%%%%%%%%%%%%%%%%%%%%%%%%%%%%%%%%%%%%%%%%%%%%%%%%%%%%%%%%%%%%%%%%%%%%%%
function [xfo, yfo] =  filter(u, Col)

lb1 = line_buffer1(u, Col);
lb2 = line_buffer2(lb1, Col);

ud1 = filterdelay1(u);
ud2 = filterdelay2(ud1);

lb1d1 = filterdelay3(lb1);
lb1d2 = filterdelay4(lb1d1);

lb2d1 = filterdelay5(lb2);
lb2d2 = filterdelay6(lb2d1);

xfo = xf(u, ud1, ud2, lb2, lb2d1, lb2d2);
yfo = yf(ud2, u, lb1d2, lb1, lb2d2, lb2);

end

%%%%%%%%%%%%%%%%%%%%%%%%%%%%%%%%%%%%%%%%%%%%%%%%%%%%%%%%%%%%%%%%%%%%%%%%%%%
% Compute x gradient
%%%%%%%%%%%%%%%%%%%%%%%%%%%%%%%%%%%%%%%%%%%%%%%%%%%%%%%%%%%%%%%%%%%%%%%%%%%
function xf_out = xf(u, xd1, xd2, lb2, zd1, zd2)
c2 = fi(2, 1,3,0, fimath(u));

t1 = fi(xd1 * c2, 1,10,0, fimath(u));
a1 = fi(u + t1 + xd2, 1,11,0, fimath(u));
pa1 = filterdelay7(a1);

t1 = fi(zd1 * c2, 1,10,0, fimath(u));
a2 = fi(lb2 + t1 + zd2, 1,11,0, fimath(u));
pa2 = filterdelay8(a2);

xf_out = fi(pa1 - pa2, 1,12,0, fimath(u));

end

%%%%%%%%%%%%%%%%%%%%%%%%%%%%%%%%%%%%%%%%%%%%%%%%%%%%%%%%%%%%%%%%%%%%%%%%%%%
% Compute y gradient
%%%%%%%%%%%%%%%%%%%%%%%%%%%%%%%%%%%%%%%%%%%%%%%%%%%%%%%%%%%%%%%%%%%%%%%%%%%
function yf_out = yf(xd2, u, yd2, lb1, zd2, lb2)
t = fi(xd2 - u, 1,11,0, fimath(u));
pa1 = filterdelay9(t);

t = fi(yd2 - lb1, 1,11,0, fimath(u));
c2 = fi(2, 1,3,0, fimath(u));
a2 = fi(c2 * t, 1,11,0, fimath(u));
pa2 = filterdelay10(a2);

t = fi(zd2 - lb2, 1,11,0, fimath(u));
pa3 = filterdelay11(t);

yf_out = fi(pa1 + pa2 + pa3, 1,13,0, fimath(u));

end

%%%%%%%%%%%%%%%%%%%%%%%%%%%%%%%%%%%%%%%%%%%%%%%%%%%%%%%%%%%%%%%%%%%%%%%%%%%
% Line Buffers %
%%%%%%%%%%%%%%%%%%%%%%%%%%%%%%%%%%%%%%%%%%%%%%%%%%%%%%%%%%%%%%%%%%%%%%%%%%%
function y = line_buffer1(u, N)
persistent u_d ctr;
if isempty(u_d)
    u_d = fi(zeros(1,N), numerictype(u), fimath(u));
    ctr = uint8(1);
end

y = u_d(ctr);
u_d(ctr) = u;

if ctr == N
    ctr = uint8(1);
else
    ctr = ctr + 1;
end
end

function y = line_buffer2(u, N)
persistent u_d ctr;
if isempty(u_d)
    u_d = fi(zeros(1,N), numerictype(u), fimath(u));
    ctr = uint8(1);
end

y = u_d(ctr);
u_d(ctr) = u;

if ctr == N
    ctr = uint8(1);
else
    ctr = ctr + 1;
end
end


%%%%%%%%%%%%%%%%%%%%%%%%%%%%%%%%%%%%%%%%%%%%%%%%%%%%%%%%%%%%%%%%%%%%%%%%%%%
% Filter Delays %
%%%%%%%%%%%%%%%%%%%%%%%%%%%%%%%%%%%%%%%%%%%%%%%%%%%%%%%%%%%%%%%%%%%%%%%%%%%

function y = filterdelay1(u)
persistent u_d;
if isempty(u_d)
    u_d = fi(0, numerictype(u), fimath(u));
end
y = u_d;
u_d = u;
end

function y = filterdelay2(u)
persistent u_d;
if isempty(u_d)
    u_d = fi(0, numerictype(u), fimath(u));
end
y = u_d;
u_d = u;
end

function y = filterdelay3(u)
persistent u_d;
if isempty(u_d)
    u_d = fi(0, numerictype(u), fimath(u));
end
y = u_d;
u_d = u;
end

function y = filterdelay4(u)
persistent u_d;
if isempty(u_d)
    u_d = fi(0, numerictype(u), fimath(u));
end
y = u_d;
u_d = u;
end

function y = filterdelay5(u)
persistent u_d;
if isempty(u_d)
    u_d = fi(0, numerictype(u), fimath(u));
end
y = u_d;
u_d = u;
end

function y = filterdelay6(u)
persistent u_d;
if isempty(u_d)
    u_d = fi(0, numerictype(u), fimath(u));
end
y = u_d;
u_d = u;
end

function y = filterdelay7(u)
persistent u_d;
if isempty(u_d)
    u_d = fi(0, numerictype(u), fimath(u));
end
y = u_d;
u_d = u;
end

function y = filterdelay8(u)
persistent u_d;
if isempty(u_d)
    u_d = fi(0, numerictype(u), fimath(u));
end
y = u_d;
u_d = u;
end

function y = filterdelay9(u)
persistent u_d;
if isempty(u_d)
    u_d = fi(0, numerictype(u), fimath(u));
end
y = u_d;
u_d = u;
end

function y = filterdelay10(u)
persistent u_d;
if isempty(u_d)
    u_d = fi(0, numerictype(u), fimath(u));
end
y = u_d;
u_d = u;
end

function y = filterdelay11(u)
persistent u_d;
if isempty(u_d)
    u_d = fi(0, numerictype(u), fimath(u));
end
y = u_d;
u_d = u;
end

function y = filterdelay12(u)
persistent u_d;
if isempty(u_d)
    u_d = fi(0, numerictype(u), fimath(u));
end
y = u_d;
u_d = u;
end

function y = filterdelay13(u)
persistent u_d;
if isempty(u_d)
    u_d = fi(0, numerictype(u), fimath(u));
end
y = u_d;
u_d = u;
end

function y = filterdelay14(u)
persistent u_d;
if isempty(u_d)
    u_d = false;
end
y = u_d;
u_d = u;
end

== matlab function eml_hdl_design_patterns/Counters/counter_mod3 ==
  settings: fimath=|
      | fimath(...
      | 'RoundMode', 'floor',...
      | 'OverflowMode', 'saturate',...
      | 'ProductMode', 'FullPrecision', 'ProductWordLength', 32,...
      | 'SumMode', 'FullPrecision', 'SumWordLength', 32,...
      | 'CastBeforeSum', true)
  data: clear input boolean; count output size=1
function count = fcn(clear)

% Count 0, 1, 2, 0, 1, 2

% This counter is configured to rollover.  If this is
% not desirable set result_fm 'OverflowMode' to 'saturate'.

result_nt = numerictype(0,8,0);
result_fm = fimath('OverflowMode', 'wrap', 'RoundMode', 'floor');

persistent count_reg;
if isempty(count_reg)
    count_reg = fi(0, result_nt, result_fm);
end

count = count_reg;

if clear
    count_reg = fi(0, result_nt, result_fm);
else
    t = fi(count_reg + 1, result_nt, result_fm);

    if (t <= fi(2, 0, 2, 0))
        count_reg = fi(t, result_nt, result_fm);
    else
        count_reg = fi(0, result_nt, result_fm);
    end    
end

== matlab function eml_hdl_design_patterns/Word Twiddlers/Integer to Bits/MATLAB Function ==
  data: u input size=1; y output; maxWordLength parameter size=1
function y = integerToBits(u,maxWordLength)
    assert(isfi(u) && isfixed(u) && isscalar(u) && isreal(u));
    assert(u.WordLength <= maxWordLength)
    y = zeros(1,maxWordLength,'like',fi([],0,1,0));
    coder.unroll
    for k = 1:u.WordLength
        y(k) = bitsliceget(u, k, k);
    end
end

== matlab function eml_hdl_design_patterns/Word Twiddlers/Bits to Integer ==
  data: u input; y output
function y = bitsToInteger(u)
    assert(isfi(u) && isfixed(u) && isvector(u) && isreal(u));
    w = length(u);
    y = fi(0,0,w,0);
    coder.unroll
    for k = 1:w
        y = bitset(y, k, u(k));
    end
end

== matlab function eml_hdl_design_patterns/Signal Analysis/conv_input_side ==
  settings: fimath=|
      | fimath(...
      | 'RoundMode', 'floor',...
      | 'OverflowMode', 'wrap',...
      | 'ProductMode', 'FullPrecision', 'ProductWordLength', 32,...
      | 'SumMode', 'FullPrecision', 'SumWordLength', 32,...
      | 'CastBeforeSum', true)
  data: u input fixdt(0,6,2) size=80; y output; h input fixdt(0,6,2) size=30
function y = fcn(u, h)

% Convolution: on the input side
% This first viewpoint of convolution is based 
% on the fundamental concept of DSP: 
% decompose the input, pass the components through 
% the system, and synthesize the output. In this example, 
% each of the nine samples in the input signal will 
% contribute a scaled and shifted version of the 
% impulse response to the output signal. 


% y has to be fully specified before indexing into it.
%  length(y) == 112, typeof(y) == ufix12_En6

y = fi(zeros(1, 110), 0, 12, 6, fimath(u));


for ii=1:80
    for jj=1:30
        kk = ii+jj;
        % multiply and truncate
        mul_t = fi(u(ii)*h(jj), 0, 12, 4);
        % accumulate and truncate
        acc_t = fi(y(kk)+ mul_t, 0, 12, 4);
        % update output
        y(kk) = acc_t;
    end
end

== matlab function eml_hdl_design_patterns/Word Twiddlers/flip_vector ==
  settings: fimath=|
      | fimath(...
      | 'RoundMode', 'floor',...
      | 'OverflowMode', 'wrap',...
      | 'ProductMode', 'FullPrecision', 'ProductWordLength', 32,...
      | 'SumMode', 'FullPrecision', 'SumWordLength', 32,...
      | 'CastBeforeSum', true)
  data: u input fixdt(0,6,1) size=[1 4]; y output
function y = fcn(u)

y = u(:,end:-1:1)';

== matlab function eml_hdl_design_patterns/Converters/gray2bin_blk ==
  settings: fimath=|
      | fimath(...
      | 'RoundMode', 'nearest',...
      | 'OverflowMode', 'saturate',...
      | 'ProductMode', 'FullPrecision', 'ProductWordLength', 128,...
      | 'SumMode', 'FullPrecision', 'SumWordLength', 128,...
      | 'CastBeforeSum', true)
  data: g2 input boolean; g1 input boolean; g0 input boolean size=1; b2 output boolean size=1; b1 output boolean; b0 output boolean
function [b2, b1, b0] = fcn(g2, g1, g0)

% Definition: An ordering of 2n binary numbers such that only one bit 
% changes from one entry to the next. Gray codes for 4 or more bits 
% are not unique, even allowing for permutation or inversion of bits. 

ng2 = ~g2;
ng1 = ~g1;
ng0 = ~g0;

b2 = (g2 & g1 & ng0)  | (g2 & g1 & g0)   | (g2 & ng1 & g0) | (g2 & ng1 & ng0);
b1 = (ng2 & g1 & g0)  | (ng2 & g1 & ng0) | (g2 & ng1 & g0) | (g2 & ng1 & ng0);
b0 = (ng2 & ng1 & g0) | (ng2 & g1 & ng0) | (g2 & g1 & g0)  | (g2 & ng1 & ng0);

== matlab function eml_hdl_design_patterns/Register Files/singleport_regfile ==
  settings: fimath=|
      | fimath(...
      | 'RoundMode', 'nearest',...
      | 'OverflowMode', 'saturate',...
      | 'ProductMode', 'FullPrecision', 'ProductWordLength', 128,...
      | 'SumMode', 'FullPrecision', 'SumWordLength', 128,...
      | 'CastBeforeSum', true)
  data: rdwr input boolean; addr input int8; datain input fixdt(0,23,0) size=1; dataout output fixdt(0,23,0) size=1
function dataout = fcn(rdwr, addr, datain)
% rdwr is a control signal;
% if rdwr == 1 then register file will be read else written
% when dataout is same as datain in write mode

% this block shows how to conver zero based address into one based 
% matlab indexing of vectors


persistent regfile;
if isempty(regfile)
    regfile = fi(zeros(64, 1), 0, 23, 0);
end

if (rdwr)
    dataout = regfile(addr+1);
else
    regfile(addr+1) = datain;
    dataout = datain;
end
